simulink model "lab6_task1"  (R2024b)
settings: Solver=ode45  StartTime=0.0  StopTime=5.0  MaxStep=0.01  RelTol=1e-3
settings Model: Creator=Beanie  LastModifiedBy=Beanie

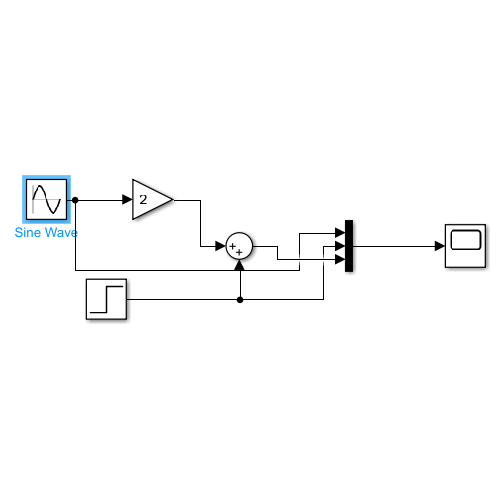
[thumbnail: Simulink's stored preview of the top-level diagram]
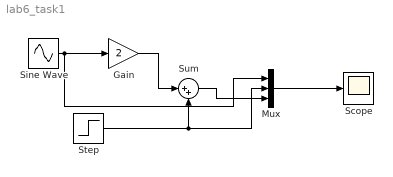
== system lab6_task1 ==
  Gain : Gain  Gain=2
  Mux : Mux  Inputs=3
  Scope : Scope
  Sine Wave : Sin  Frequency=4*pi  SampleTime=0
  Step : Step  SampleTime=0
  Sum : Sum  Inputs=|++
  wires:
  Sine Wave/1 -> Mux/1, Gain/1
  Step/1 -> Mux/2, Sum/2
  Gain/1 -> Sum/1
  Sum/1 -> Mux/3
  Mux/1 -> Scope/1
